simulink model "AnkelBot"  (R2026b)
settings: Solver=FixedStepDiscrete  StopTime=600  FixedStep=0.1
settings Model: Creator=ASOS  LastModifiedBy=ASOS

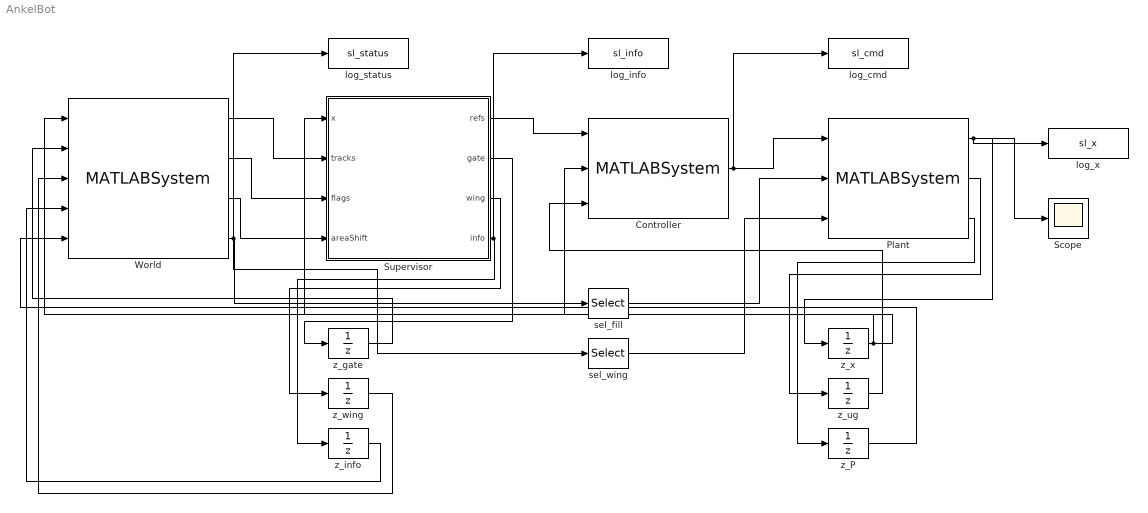
== system AnkelBot ==
  Controller : MATLABSystem  System=ankel.sys.ControllerBlock  SampleTime=0.1  SimulateUsing=Interpreted execution
      mask Type: ankel.sys.ControllerBlock
  Plant : MATLABSystem  System=ankel.sys.PlantBlock  Current=[0 0]  SampleTime=0.1  SimulateUsing=Interpreted execution
      mask Type: ankel.sys.PlantBlock
  Scope : Scope
  Supervisor : Stateflow chart  TreatAsAtomicUnit=on
  World : MATLABSystem  System=ankel.sys.WorldBlock  Scenario=mixed  SampleTime=0.1  SimulateUsing=Interpreted execution
      mask Type: ankel.sys.WorldBlock
  log_cmd : ToWorkspace  VariableName=sl_cmd  SampleTime=-1
  log_info : ToWorkspace  VariableName=sl_info  SampleTime=-1
  log_status : ToWorkspace  VariableName=sl_status  SampleTime=-1
  log_x : ToWorkspace  VariableName=sl_x  SampleTime=-1
  sel_fill : Selector  InputPortWidth=6  IndexOptions=Index vector (dialog)  Indices=1  OutputSizes=1
  sel_wing : Selector  InputPortWidth=6  IndexOptions=Index vector (dialog)  Indices=[2 3]  OutputSizes=1
  z_P : UnitDelay  InitialCondition=25  SampleTime=0.1
  z_gate : UnitDelay  SampleTime=0.1
  z_info : UnitDelay  InitialCondition=[1 0]  SampleTime=0.1
  z_ug : UnitDelay  SampleTime=0.1
  z_wing : UnitDelay  InitialCondition=[0.698131700797732 0.698131700797732]  SampleTime=0.1
  z_x : UnitDelay  InitialCondition=zeros(6,1)  SampleTime=0.1
  wires:
  World/1 -> Supervisor/2(tracks)
  World/2 -> Supervisor/3(flags)
  World/3 -> Supervisor/4(areaShift)
  Supervisor/1(refs) -> Controller/1
  Controller/1 -> Plant/1, log_cmd/1
  Plant/1 -> z_x/1, log_x/1, Scope/1
  Plant/2 -> z_ug/1
  Plant/3 -> z_P/1
  z_x/1 -> World/1, Supervisor/1(x), Controller/2
  z_ug/1 -> Controller/3
  z_P/1 -> World/5
  Supervisor/2(gate) -> z_gate/1
  Supervisor/3(wing) -> z_wing/1
  Supervisor/4(info) -> z_info/1, log_info/1
  z_gate/1 -> World/2
  z_wing/1 -> World/3
  z_info/1 -> World/4
  World/4 -> sel_fill/1, sel_wing/1, log_status/1
  sel_fill/1 -> Plant/2
  sel_wing/1 -> Plant/3

== stateflow chart AnkelBot/Supervisor ==
  settings: updateMethod=DISCRETE  sampleTime=0.1
  state MISSION
    entry:
    coder.extrinsic('sfScan', 'sfEntry', 'sfOut');
    st = 1; ts = 0; gp = 0; first = 1; mem = [1 0 0 -1 0];
    v = zeros(1, 17);
    v = sfScan(st, ts, gp, 0, 99, mem(5), x, tracks, flags, areaShift);
    during:
    coder.extrinsic('sfScan', 'sfEntry', 'sfOut');
    first = 0;
    v = sfScan(st, ts, gp, v(15), v(16), mem(5), x, tracks, flags, areaShift);
    state ACTIVE
      state NORMAL
        state SEARCH
          entry:
          coder.extrinsic('sfScan', 'sfEntry', 'sfOut');
          st = 1; ts = 0;
          mem = sfEntry(st, mem, v, x);
          r = sfOut(st, ts, mem, v, x, areaShift);
          refs = r(1:3); gate = r(4); wing = r(5:6);
          mem = r(7:11); gp = r(4); info = [st ts];
          during:
          coder.extrinsic('sfScan', 'sfEntry', 'sfOut');
          ts = ts + v(17);
          r = sfOut(st, ts, mem, v, x, areaShift);
          refs = r(1:3); gate = r(4); wing = r(5:6);
          mem = r(7:11); gp = r(4); info = [st ts];
        state APPROACH
          entry:
          coder.extrinsic('sfScan', 'sfEntry', 'sfOut');
          st = 2; ts = 0;
          mem = sfEntry(st, mem, v, x);
          r = sfOut(st, ts, mem, v, x, areaShift);
          refs = r(1:3); gate = r(4); wing = r(5:6);
          mem = r(7:11); gp = r(4); info = [st ts];
          during:
          coder.extrinsic('sfScan', 'sfEntry', 'sfOut');
          ts = ts + v(17);
          r = sfOut(st, ts, mem, v, x, areaShift);
          refs = r(1:3); gate = r(4); wing = r(5:6);
          mem = r(7:11); gp = r(4); info = [st ts];
        state AVOID
          entry:
          coder.extrinsic('sfScan', 'sfEntry', 'sfOut');
          st = 3; ts = 0;
          mem = sfEntry(st, mem, v, x);
          r = sfOut(st, ts, mem, v, x, areaShift);
          refs = r(1:3); gate = r(4); wing = r(5:6);
          mem = r(7:11); gp = r(4); info = [st ts];
          during:
          coder.extrinsic('sfScan', 'sfEntry', 'sfOut');
          ts = ts + v(17);
          r = sfOut(st, ts, mem, v, x, areaShift);
          refs = r(1:3); gate = r(4); wing = r(5:6);
          mem = r(7:11); gp = r(4); info = [st ts];
        state RETURN
          entry:
          coder.extrinsic('sfScan', 'sfEntry', 'sfOut');
          st = 5; ts = 0;
          mem = sfEntry(st, mem, v, x);
          r = sfOut(st, ts, mem, v, x, areaShift);
          refs = r(1:3); gate = r(4); wing = r(5:6);
          mem = r(7:11); gp = r(4); info = [st ts];
          during:
          coder.extrinsic('sfScan', 'sfEntry', 'sfOut');
          ts = ts + v(17);
          r = sfOut(st, ts, mem, v, x, areaShift);
          refs = r(1:3); gate = r(4); wing = r(5:6);
          mem = r(7:11); gp = r(4); info = [st ts];
        (default) -> (junction 31)
        (junction 31) -> APPROACH [order 3] : [first > 0.5 && v(14) == 2]
        (junction 31) -> SEARCH [order 4]
        (junction 31) -> AVOID [order 2] : [first > 0.5 && v(14) == 3]
        (junction 31) -> RETURN [order 1] : [first > 0.5 && v(14) == 5]
        SEARCH -> APPROACH [order 1] : [v(14) == 2]
        APPROACH -> SEARCH [order 1] : [v(14) == 1]
        AVOID -> SEARCH [order 1] : [v(14) == 1]
        SEARCH -> AVOID [order 2] : [v(14) == 3]
        RETURN -> SEARCH [order 1] : [v(14) == 1]
        SEARCH -> RETURN [order 3] : [v(14) == 5]
        APPROACH -> AVOID [order 2] : [v(14) == 3]
        AVOID -> APPROACH [order 2] : [v(14) == 2]
        RETURN -> APPROACH [order 2] : [v(14) == 2]
        APPROACH -> RETURN [order 3] : [v(14) == 5]
        AVOID -> RETURN [order 3] : [v(14) == 5]
        RETURN -> AVOID [order 3] : [v(14) == 3]
      state BACKOFF
        entry:
        coder.extrinsic('sfScan', 'sfEntry', 'sfOut');
        st = 4; ts = 0;
        mem = sfEntry(st, mem, v, x);
        r = sfOut(st, ts, mem, v, x, areaShift);
        refs = r(1:3); gate = r(4); wing = r(5:6);
        mem = r(7:11); gp = r(4); info = [st ts];
        during:
        coder.extrinsic('sfScan', 'sfEntry', 'sfOut');
        ts = ts + v(17);
        r = sfOut(st, ts, mem, v, x, areaShift);
        refs = r(1:3); gate = r(4); wing = r(5:6);
        mem = r(7:11); gp = r(4); info = [st ts];
      state DOCKED
        entry:
        coder.extrinsic('sfScan', 'sfEntry', 'sfOut');
        st = 6; ts = 0;
        mem = sfEntry(st, mem, v, x);
        r = sfOut(st, ts, mem, v, x, areaShift);
        refs = r(1:3); gate = r(4); wing = r(5:6);
        mem = r(7:11); gp = r(4); info = [st ts];
        during:
        coder.extrinsic('sfScan', 'sfEntry', 'sfOut');
        ts = ts + v(17);
        r = sfOut(st, ts, mem, v, x, areaShift);
        refs = r(1:3); gate = r(4); wing = r(5:6);
        mem = r(7:11); gp = r(4); info = [st ts];
      (default) -> NORMAL
      (junction 27) -> BACKOFF
      BACKOFF -> (junction 27) [order 1] : [v(12) < 0.5 && v(8) > 0.5]
      (junction 26) -> SEARCH [order 5]
      (junction 26) -> APPROACH [order 4] : [v(14) == 2]
      NORMAL -> BACKOFF [order 1] : [v(8) > 0.5]
      BACKOFF -> (junction 26) [order 2] : [v(12) < 0.5]
      DOCKED -> BACKOFF [order 1] : [v(13) < 0.5 && v(8) > 0.5]
      (junction 26) -> DOCKED [order 1] : [v(9) > 0.5 && v(10) > 0.5]
      (junction 26) -> AVOID [order 3] : [v(14) == 3]
      (junction 26) -> RETURN [order 2] : [v(14) == 5]
      NORMAL -> DOCKED [order 2] : [v(9) > 0.5 && v(10) > 0.5]
      DOCKED -> (junction 26) [order 2] : [v(13) < 0.5]
    state FAILSAFE
      entry:
      coder.extrinsic('sfScan', 'sfEntry', 'sfOut');
      st = 7; ts = 0;
      mem = sfEntry(st, mem, v, x);
      r = sfOut(st, ts, mem, v, x, areaShift);
      refs = r(1:3); gate = r(4); wing = r(5:6);
      mem = r(7:11); gp = r(4); info = [st ts];
      during:
      coder.extrinsic('sfScan', 'sfEntry', 'sfOut');
      ts = ts + v(17);
      r = sfOut(st, ts, mem, v, x, areaShift);
      refs = r(1:3); gate = r(4); wing = r(5:6);
      mem = r(7:11); gp = r(4); info = [st ts];
    (default) -> ACTIVE
    FAILSAFE -> ACTIVE : [v(11) > 0.5]
    ACTIVE -> FAILSAFE : [v(11) < 0.5]
  (default) -> MISSION
  data: x input double size=6; tracks input double size=[8 5]; flags input double size=5; areaShift input double size=2; refs output double size=[1 3]; gate output double size=1; wing output double size=[1 2]; info output double size=[1 2]; v local double size=[1 17]; mem local double size=[1 5]; r local double size=[1 11]; st local double size=1; ts local double size=1; gp local double size=1; first local double size=1
